simulink model "gnc_ImplementManager"  (R2026b)
settings: Solver=VariableStepAuto
values from neighbouring files (symbols this model uses):
  Ts = prm.Ts    [gnc_missionFSM.m]    (also in gnc_mpcPlantUpdate.m)
undefined symbols (not defined in the file or in its folder): AutoSub, deck_height_cmd, GncState, ImplementType, mower_enable, mower_speed_cmd, P, spray_enable, spray_flow_cmd, spray_section_mask, tiller_depth_cmd, tiller_enable, tiller_speed_cmd
libraries: simulink x11
settings Model: Creator=aomar  LastModifiedBy=aomar

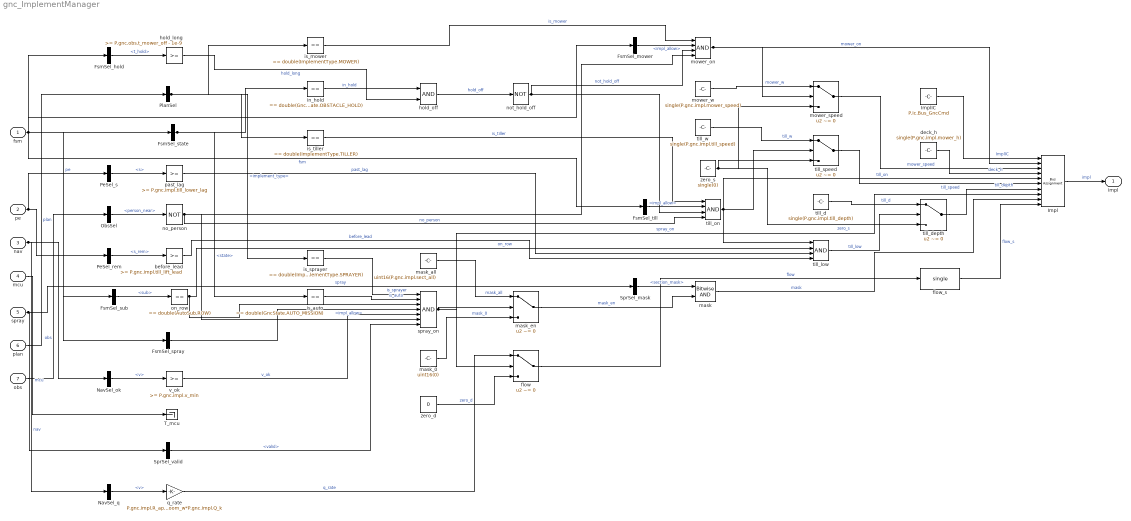
== system gnc_ImplementManager ==
  fsm : Inport  OutDataTypeStr=Bus: Bus_FsmOut  SampleTime=Ts.gnc
  pe : Inport  Port=2  OutDataTypeStr=Bus: Bus_PathError  SampleTime=Ts.gnc
  nav : Inport  Port=3  OutDataTypeStr=Bus: Bus_NavCond  SampleTime=Ts.gnc
  mcu : Inport  Port=4  OutDataTypeStr=Bus: Bus_McuStatus  SampleTime=Ts.gnc
  spray : Inport  Port=5  OutDataTypeStr=Bus: Bus_SprayDemand  SampleTime=Ts.gnc
  plan : Inport  Port=6  OutDataTypeStr=Bus: Bus_MissionPlan
  obs : Inport  Port=7  OutDataTypeStr=Bus: Bus_ObsFlags  SampleTime=Ts.gnc
  FsmSel_hold : BusSelector  OutputSignals=t_hold
  FsmSel_mower : BusSelector  OutputSignals=impl_allow
  FsmSel_spray : BusSelector  OutputSignals=impl_allow
  FsmSel_state : BusSelector  OutputSignals=state
  FsmSel_sub : BusSelector  OutputSignals=sub
  FsmSel_till : BusSelector  OutputSignals=impl_allow
  Impl : BusAssignment  AssignedSignals=mower_enable,mower_speed_cmd,deck_height_cmd,tiller_enable,tiller_speed_cmd,tiller_depth_cmd,spray_enable,spray_section_mask,spray_flow_cmd
  ImplIC : Constant  Value=P.ic.Bus_GncCmd  OutDataTypeStr=Bus: Bus_GncCmd  SampleTime=Ts.gnc
  NavSel_ok : BusSelector  OutputSignals=v
  NavSel_q : BusSelector  OutputSignals=v
  ObsSel : BusSelector  OutputSignals=person_near
  PeSel_rem : BusSelector  OutputSignals=s_rem
  PeSel_s : BusSelector  OutputSignals=s
  PlanSel : BusSelector  OutputSignals=implement_type
  SprSel_mask : BusSelector  OutputSignals=section_mask
  SprSel_valid : BusSelector  OutputSignals=valid
  T_mcu : Terminator
  before_lead : simulink/Logic and Bit Operations/Compare To Constant  relop=>=  const=P.gnc.impl.till_lift_lead  OutDataTypeStr=boolean
  deck_h : Constant  Value=single(P.gnc.impl.mower_h)  OutDataTypeStr=single  SampleTime=Ts.gnc
  flow : Switch  Criteria=u2 ~= 0  SaturateOnIntegerOverflow=off  InputSameDT=off
  flow_s : DataTypeConversion  OutDataTypeStr=single  RndMeth=Nearest
  hold_long : simulink/Logic and Bit Operations/Compare To Constant  relop=>=  const=P.gnc.obs.t_mower_off - 1e-9  OutDataTypeStr=boolean
  hold_off : Logic  AllPortsSameDT=off  OutDataTypeStr=boolean
  in_hold : simulink/Logic and Bit Operations/Compare To Constant  relop===  const=double(GncState.OBSTACLE_HOLD)  OutDataTypeStr=boolean
  is_auto : simulink/Logic and Bit Operations/Compare To Constant  relop===  const=double(GncState.AUTO_MISSION)  OutDataTypeStr=boolean
  is_mower : simulink/Logic and Bit Operations/Compare To Constant  relop===  const=double(ImplementType.MOWER)  OutDataTypeStr=boolean
  is_sprayer : simulink/Logic and Bit Operations/Compare To Constant  relop===  const=double(ImplementType.SPRAYER)  OutDataTypeStr=boolean
  is_tiller : simulink/Logic and Bit Operations/Compare To Constant  relop===  const=double(ImplementType.TILLER)  OutDataTypeStr=boolean
  mask : simulink/Logic and Bit Operations/Bitwise Operator  logicop=AND  UseBitMask=off  NumInputPorts=2  BitMask=bin2dec('11011001')  BitMaskRealWorld=Stored Integer
  mask_0 : Constant  Value=uint16(0)  OutDataTypeStr=uint16  SampleTime=Ts.gnc
  mask_all : Constant  Value=uint16(P.gnc.impl.sect_all)  OutDataTypeStr=uint16  SampleTime=Ts.gnc
  mask_en : Switch  Criteria=u2 ~= 0  SaturateOnIntegerOverflow=off  InputSameDT=off
  mower_on : Logic  Inputs=4  AllPortsSameDT=off  OutDataTypeStr=boolean
  mower_speed : Switch  Criteria=u2 ~= 0  SaturateOnIntegerOverflow=off  InputSameDT=off
  mower_w : Constant  Value=single(P.gnc.impl.mower_speed)  OutDataTypeStr=single  SampleTime=Ts.gnc
  no_person : Logic  Operator=NOT  Inputs=1  AllPortsSameDT=off  OutDataTypeStr=boolean
  not_hold_off : Logic  Operator=NOT  Inputs=1  AllPortsSameDT=off  OutDataTypeStr=boolean
  on_row : simulink/Logic and Bit Operations/Compare To Constant  relop===  const=double(AutoSub.ROW)  OutDataTypeStr=boolean
  past_lag : simulink/Logic and Bit Operations/Compare To Constant  relop=>=  const=P.gnc.impl.till_lower_lag  OutDataTypeStr=boolean
  q_rate : Gain  Gain=P.gnc.impl.R_app*P.gnc.impl.boom_w*P.gnc.impl.Q_k
  spray_on : Logic  Inputs=7  AllPortsSameDT=off  OutDataTypeStr=boolean
  till_d : Constant  Value=single(P.gnc.impl.till_depth)  OutDataTypeStr=single  SampleTime=Ts.gnc
  till_depth : Switch  Criteria=u2 ~= 0  SaturateOnIntegerOverflow=off  InputSameDT=off
  till_low : Logic  Inputs=4  AllPortsSameDT=off  OutDataTypeStr=boolean
  till_on : Logic  Inputs=4  AllPortsSameDT=off  OutDataTypeStr=boolean
  till_speed : Switch  Criteria=u2 ~= 0  SaturateOnIntegerOverflow=off  InputSameDT=off
  till_w : Constant  Value=single(P.gnc.impl.till_speed)  OutDataTypeStr=single  SampleTime=Ts.gnc
  v_ok : simulink/Logic and Bit Operations/Compare To Constant  relop=>=  const=P.gnc.impl.v_min  OutDataTypeStr=boolean
  zero_d : Constant  Value=0  OutDataTypeStr=double  SampleTime=Ts.gnc
  zero_s : Constant  Value=single(0)  OutDataTypeStr=single  SampleTime=Ts.gnc
  impl : Outport  OutDataTypeStr=Bus: Bus_GncCmd
  wires:
  mcu/1 -> T_mcu/1  "mcu"
  plan/1 -> PlanSel/1  "plan"
  FsmSel_hold/1 -> hold_long/1  "<t_hold>"
  PeSel_s/1 -> past_lag/1  "<s>"
  ObsSel/1 -> no_person/1  "<person_near>"
  PeSel_rem/1 -> before_lead/1  "<s_rem>"
  NavSel_ok/1 -> v_ok/1  "<v>"
  NavSel_q/1 -> q_rate/1  "<v>"
  FsmSel_sub/1 -> on_row/1  "<sub>"
  PlanSel/1 -> is_sprayer/1, is_mower/1, is_tiller/1  "<implement_type>"
  FsmSel_spray/1 -> spray_on/4  "<impl_allow>"
  SprSel_valid/1 -> spray_on/7  "<valid>"
  FsmSel_state/1 -> is_auto/1, in_hold/1  "<state>"
  hold_long/1 -> hold_off/2  "hold_long"
  past_lag/1 -> till_low/3  "past_lag"
  no_person/1 -> mower_on/4, spray_on/6, till_on/4  "no_person"
  before_lead/1 -> till_low/4  "before_lead"
  v_ok/1 -> spray_on/5  "v_ok"
  q_rate/1 -> flow/1  "q_rate"
  on_row/1 -> till_low/2, spray_on/3  "on_row"
  is_mower/1 -> mower_on/1  "is_mower"
  in_hold/1 -> hold_off/1  "in_hold"
  is_tiller/1 -> till_on/1  "is_tiller"
  is_sprayer/1 -> spray_on/1  "is_sprayer"
  is_auto/1 -> spray_on/2  "is_auto"
  hold_off/1 -> not_hold_off/1  "hold_off"
  mask_all/1 -> mask_en/1  "mask_all"
  spray_on/1 -> Impl/8, flow/2, mask_en/2  "spray_on"
  mask_0/1 -> mask_en/3  "mask_0"
  zero_d/1 -> flow/3  "zero_d"
  not_hold_off/1 -> till_on/3, mower_on/3  "not_hold_off"
  mask_en/1 -> mask/2  "mask_en"
  flow/1 -> flow_s/1  "flow"
  FsmSel_mower/1 -> mower_on/2  "<impl_allow>"
  SprSel_mask/1 -> mask/1  "<section_mask>"
  FsmSel_till/1 -> till_on/2  "<impl_allow>"
  mower_on/1 -> Impl/2, mower_speed/2  "mower_on"
  mower_w/1 -> mower_speed/1  "mower_w"
  till_w/1 -> till_speed/1  "till_w"
  zero_s/1 -> mower_speed/3, till_depth/3, till_speed/3  "zero_s"
  mask/1 -> Impl/9  "mask"
  till_on/1 -> till_speed/2, till_low/1, Impl/5  "till_on"
  till_d/1 -> till_depth/1  "till_d"
  till_low/1 -> till_depth/2  "till_low"
  mower_speed/1 -> Impl/3  "mower_speed"
  till_speed/1 -> Impl/6  "till_speed"
  ImplIC/1 -> Impl/1  "ImplIC"
  deck_h/1 -> Impl/4  "deck_h"
  till_depth/1 -> Impl/7  "till_depth"
  flow_s/1 -> Impl/10  "flow_s"
  Impl/1 -> impl/1  "impl"
  nav/1 -> NavSel_q/1, NavSel_ok/1  "nav"
  obs/1 -> ObsSel/1  "obs"
  spray/1 -> SprSel_valid/1, SprSel_mask/1  "spray"
  fsm/1 -> FsmSel_spray/1, FsmSel_sub/1, FsmSel_mower/1, FsmSel_hold/1, FsmSel_till/1, FsmSel_state/1  "fsm"
  pe/1 -> PeSel_rem/1, PeSel_s/1  "pe"
